simulink model "ARDroneTT"  (R2026a)
settings: Solver=ode1  StopTime=inf  FixedStep=sampleTime  EnableMultiTasking=on
values from neighbouring files (symbols this model uses):
  sampleTime = 0.03    [setupHover.m]    (also in setupTT.m; setupWPTracking.m = 0.065)
undefined symbols (not defined in the file or in its folder): DiscIntNeverNeededParam, Standard_Devices, UDP_Protocol
libraries: sldrtlib x3, dspnetwork x3, ARBlocks x2, simulink x1, aerolibanimutils x1
settings Model: ExtModeTrigDuration=100000  Creator=Paul  LastModifiedBy=dasos
settings DataIOCC: SignalLoggingSaveFormat=ModelDataLogs  TimeSaveName=time
settings OptimizationCC: InitFltsAndDblsToZero=on
settings DebuggingCC: UnderspecifiedInitializationDetection=Classic
settings HardwareCC: ProdBitPerLong=64.0  ProdHWDeviceType=Intel->x86-64 (Linux 64)
settings RTWCC: SystemTargetFile=sldrt.tlc  TemplateMakefile=sldrt.tmf  RTWCompilerOptimization=on  Description=Simulink Desktop Real-Time
settings CodeAppCC: MaxIdLength=95.0
settings SimulinkDesktopRealTimeCC: RealTimeExecution=kernel  ExtModeTransport=0.0  ExtModeStaticAllocSize=1000000.0  TargetLibSuffix=_sldrt.a  TargetPreCompLibLocation=C:\Program Files\MATLAB\R2026a\toolbox\sldrt\lib\win64  TargetLangStandard=C89/C90 (ANSI)  MultiwordLength=2048.0  ParMdlRefBuildCompliant=on

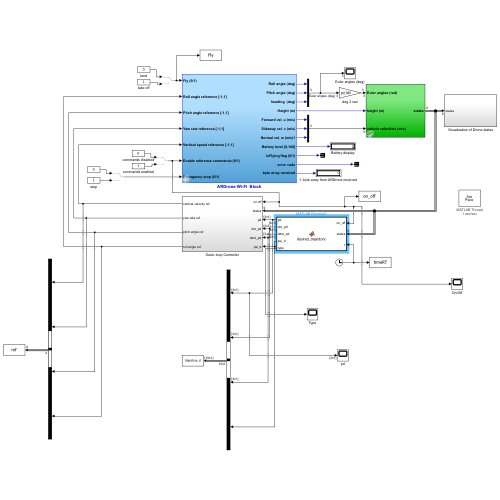
[thumbnail: Simulink's stored preview of the top-level diagram]
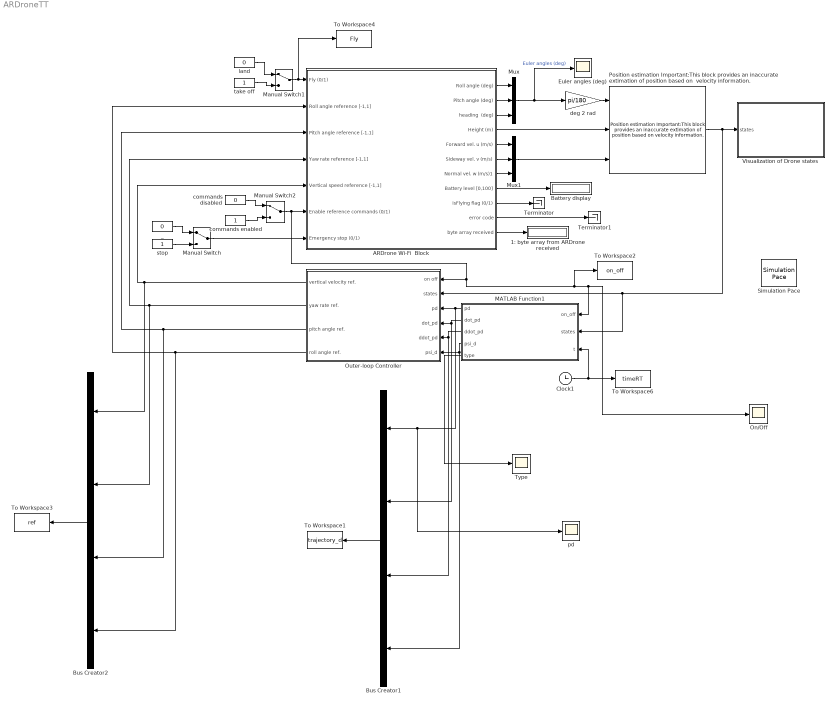
== system ARDroneTT ==
  "1: byte array from ARDrone received " : Display
  ARDrone Wi-Fi  Block : Subsystem  AncestorBlock="ARBlocks/ARDrone Wi-Fi  Block"
  Battery display : Display
  Bus Creator1 : BusCreator  Inputs=4
  Bus Creator2 : BusCreator  Inputs=4
  Clock1 : Clock
  Euler angles (deg) : Scope
      settings: ActiveDisplayYMinimum=-189.44824826717377  ActiveDisplayYMaximum=31.394250273704525  DataLoggingMaxPoints=500000
  MATLAB Function1 : MATLAB Function  TreatAsAtomicUnit=on  SystemSampleTime=sampleTime
  Manual Switch : ManualSwitch
  Manual Switch1 : ManualSwitch
  Manual Switch2 : ManualSwitch
  Mux : Mux  Inputs=3
  Mux1 : Mux  Inputs=3
  On/Off : Scope
      settings: ActiveDisplayYMinimum=-0.12499999999999997  ActiveDisplayYMaximum=1.125  DataLoggingMaxPoints=500000  DataLoggingVariableName=ScopeData13
  Outer-loop Controller : Subsystem
  "Position estimation Important:This block provides an inaccurate extimation of position based on  velocity information. " : ARBlocks/Position estimation Important:This block provides an  inaccurate extimation of position  based on  velocity information.   SystemSampleTime=-1  VariantActivationTime=update diagram  EmptyChoice=off  PassThrough=off  PassThroughVariantControl=(default)  EmptyChoiceVariantControl=(default)  AllowFlexibleInterface=on  Latency=0  AutoFrameSizeCalculation=off
  Simulation Pace : aerolibanimutils/Simulation Pace  SimulationPace=1  SleepMode=MATLAB Thread  OutputPaceError=off  SampleTime=sampleTime
  Terminator : Terminator
  Terminator1 : Terminator
  To Workspace1 : ToWorkspace  VariableName=trajectory_d  SampleTime=sampleTime
  To Workspace2 : ToWorkspace  VariableName=on_off  SampleTime=sampleTime
  To Workspace3 : ToWorkspace  VariableName=ref  SampleTime=sampleTime
  To Workspace4 : ToWorkspace  VariableName=Fly  SampleTime=sampleTime
  To Workspace6 : ToWorkspace  VariableName=timeRT  SampleTime=sampleTime
  Type : Scope
      settings: ActiveDisplayYMinimum=-1.25  ActiveDisplayYMaximum=1.25  DataLoggingMaxPoints=500000  DataLoggingVariableName=ScopeData12
  Visualization of Drone states : Subsystem
  _ : Constant  Value=0
  commands disabled : Constant  Value=0
  commands enabled : Constant
  deg 2 rad : Gain  Gain=pi/180
  land : Constant  Value=0
  pd : Scope
      settings: ActiveDisplayYMinimum=-1.25  ActiveDisplayYMaximum=1.25  DataLoggingMaxPoints=500000  DataLoggingVariableName=ScopeData11
  stop : Constant
  take off : Constant
  wires:
  _/1 -> Manual Switch/1
  stop/1 -> Manual Switch/2
  land/1 -> Manual Switch1/1
  take off/1 -> Manual Switch1/2
  commands disabled/1 -> Manual Switch2/1
  commands enabled/1 -> Manual Switch2/2
  Manual Switch1/1 -> To Workspace4/1, ARDrone Wi-Fi  Block/1(Fly (0/1))
  Manual Switch2/1 -> ARDrone Wi-Fi  Block/6(Enable reference commands (0/1)), To Workspace2/1, On/Off/1, MATLAB Function1/1(on_off), Outer-loop Controller/1(on off)
  Manual Switch/1 -> ARDrone Wi-Fi  Block/7(Emergency stop (0/1))
  ARDrone Wi-Fi  Block/1(Roll angle (deg)) -> Mux/1
  ARDrone Wi-Fi  Block/2(Pitch angle (deg)) -> Mux/2
  ARDrone Wi-Fi  Block/5(Forward vel. u (m/s)) -> Mux1/1
  ARDrone Wi-Fi  Block/6(Sideway vel. v (m/s)) -> Mux1/2
  ARDrone Wi-Fi  Block/7(Normal vel. w (m/s)1) -> Mux1/3
  Mux/1 -> Euler angles (deg)/1, deg 2 rad/1  "Euler angles (deg)"
  ARDrone Wi-Fi  Block/8(Battery level [0,100]) -> Battery display/1
  "Position estimation Important:This block provides an inaccurate extimation of position based on  velocity information. "/1 -> MATLAB Function1/2(states), Outer-loop Controller/2(states), Visualization of Drone states/1(states)
  deg 2 rad/1 -> "Position estimation Important:This block provides an inaccurate extimation of position based on  velocity information. "/1
  ARDrone Wi-Fi  Block/4(Height (m)) -> "Position estimation Important:This block provides an inaccurate extimation of position based on  velocity information. "/2
  Mux1/1 -> "Position estimation Important:This block provides an inaccurate extimation of position based on  velocity information. "/3
  ARDrone Wi-Fi  Block/3(heading  (deg)) -> Mux/3
  ARDrone Wi-Fi  Block/9(isFlying flag (0/1)) -> Terminator/1
  ARDrone Wi-Fi  Block/10(error code) -> Terminator1/1
  ARDrone Wi-Fi  Block/11(byte array received) -> "1: byte array from ARDrone received "/1
  Clock1/1 -> MATLAB Function1/3(t), To Workspace6/1
  MATLAB Function1/1(pd) -> pd/1, Bus Creator1/1, Outer-loop Controller/3(pd)
  MATLAB Function1/2(dot_pd) -> Bus Creator1/2, Outer-loop Controller/4(dot_pd)
  MATLAB Function1/3(ddot_pd) -> Bus Creator1/3, Outer-loop Controller/5(ddot_pd)
  MATLAB Function1/4(psi_d) -> Bus Creator1/4, Outer-loop Controller/6(psi_d)
  Bus Creator1/1 -> To Workspace1/1
  Outer-loop Controller/3(pitch angle ref.) -> Bus Creator2/3, ARDrone Wi-Fi  Block/3(Pitch angle reference [-1,1])
  Outer-loop Controller/2(yaw rate ref.) -> Bus Creator2/2, ARDrone Wi-Fi  Block/4(Yaw rate reference [-1,1])
  Outer-loop Controller/4(roll angle ref.) -> Bus Creator2/4, ARDrone Wi-Fi  Block/2(Roll angle reference [-1,1])
  Outer-loop Controller/1(vertical velocity ref.) -> Bus Creator2/1, ARDrone Wi-Fi  Block/5(Vertical speed reference [-1,1])
  Bus Creator2/1 -> To Workspace3/1
  MATLAB Function1/5(type) -> Type/1

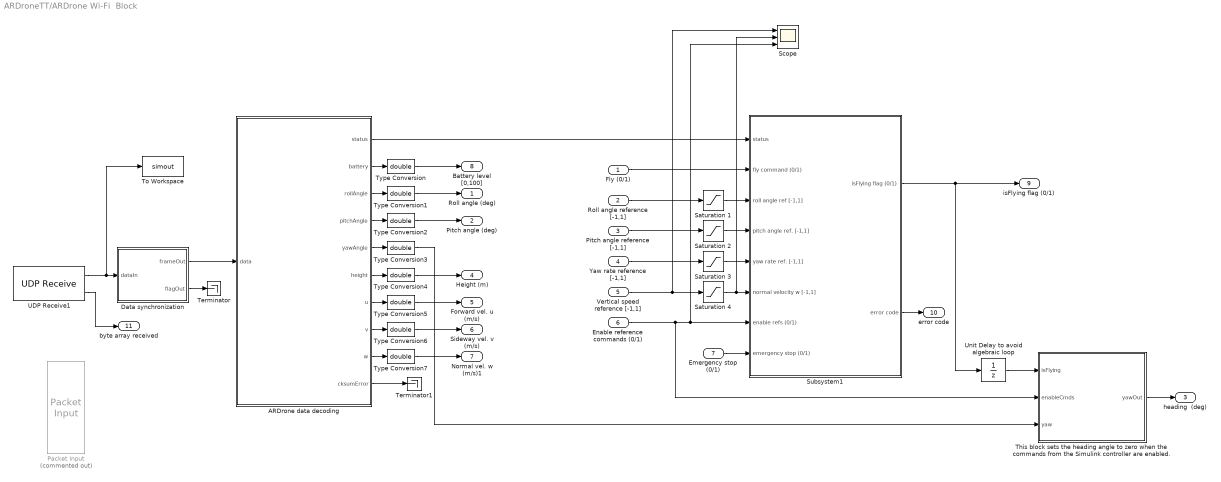
== system ARDroneTT/ARDrone Wi-Fi  Block ==
  Fly (0/1) : Inport
  Roll angle reference [-1,1] : Inport  Port=2
  Pitch angle reference [-1,1] : Inport  Port=3
  Yaw rate reference [-1,1] : Inport  Port=4
  Vertical speed reference [-1,1] : Inport  Port=5
  Enable reference commands (0/1) : Inport  Port=6
  Emergency stop (0/1) : Inport  Port=7
  ARDrone data decoding : MATLAB Function  TreatAsAtomicUnit=on
  "Data synchronization " : MATLAB Function  TreatAsAtomicUnit=on
  Packet Input : sldrtlib/Packet Input  Commented=on  SampleTime=sampleTime  MaxMissedTicks=100  ShowMissedTicks=off  YieldWhenWaiting=off  DrvName=Standard_Devices/UDP_Protocol  DrvAddress=5554  DrvOptions=[3232235777 5554]  PacketSize=500  DataTypes='500*uint8'  ShowReady=on  ShowError=off  PacketID=1  ByteOrder=1  ShowTimestamp=off
      settings: AttributesFormatString=UDP Protocol [5554]
  Saturation 1 : Saturate  UpperLimit=1  LowerLimit=-1
  Saturation 2 : Saturate  UpperLimit=1  LowerLimit=-1
  Saturation 3 : Saturate  UpperLimit=1  LowerLimit=-1
  Saturation 4 : Saturate  UpperLimit=1.5  LowerLimit=-1.5
  Scope : Scope  NumInputPorts=3
      settings: ActiveDisplayYMinimum=-0.2465  ActiveDisplayYMaximum=1.1385  DataLoggingVariableName=ScopeData2
  Subsystem1 : Subsystem
  Terminator : Terminator
  Terminator1 : Terminator
  "This block sets the heading angle to zero when the commands from the Simulink controller are enabled. " : MATLAB Function  TreatAsAtomicUnit=on
  To Workspace : ToWorkspace  VariableName=simout  SampleTime=-1
  Type Conversion{,1..7} (8 alike) : DataTypeConversion  OutDataTypeStr=double  SaturateOnIntegerOverflow=off  RndMeth=Floor
  UDP Receive1 : dspnetwork/UDP Receive  localURL='0.0.0.0'  localPort=5554  remoteURL='192.168.1.1'  remotePort=-1  recvBufferSize=8192  dims=500  signalDatatype=uint8  isComplex=off  isVarSize=off  showBlockingTime=off  blockingTime=0  sampletime=sampleTime  blockPlatform=[]
  Unit Delay to avoid algebraic loop : UnitDelay  SampleTime=-1
  Roll angle (deg) : Outport  VectorParamsAs1DForOutWhenUnconnected=off
  Pitch angle (deg) : Outport  Port=2  VectorParamsAs1DForOutWhenUnconnected=off
  heading  (deg) : Outport  Port=3  VectorParamsAs1DForOutWhenUnconnected=off
  Height (m) : Outport  Port=4  VectorParamsAs1DForOutWhenUnconnected=off
  Forward vel. u (m/s) : Outport  Port=5  VectorParamsAs1DForOutWhenUnconnected=off
  Sideway vel. v (m/s) : Outport  Port=6  VectorParamsAs1DForOutWhenUnconnected=off
  Normal vel. w (m/s)1 : Outport  Port=7  VectorParamsAs1DForOutWhenUnconnected=off
  Battery level [0,100] : Outport  Port=8  VectorParamsAs1DForOutWhenUnconnected=off
  isFlying flag (0/1) : Outport  Port=9  VectorParamsAs1DForOutWhenUnconnected=off
  error code : Outport  Port=10  VectorParamsAs1DForOutWhenUnconnected=off
  byte array received : Outport  Port=11  VectorParamsAs1DForOutWhenUnconnected=off
  wires:
  Unit Delay to avoid algebraic loop/1 -> "This block sets the heading angle to zero when the commands from the Simulink controller are enabled. "/1(isFlying)
  "Data synchronization "/2(flagOut) -> Terminator/1
  Saturation 4/1 -> Scope/2, Subsystem1/6(normal velocity w [-1,1])
  Saturation 3/1 -> Subsystem1/5(yaw rate ref. [-1,1])
  Saturation 2/1 -> Subsystem1/4(pitch angle ref. [-1,1])
  Saturation 1/1 -> Subsystem1/3(roll angle ref [-1,1])
  Fly (0/1)/1 -> Subsystem1/2(fly command (0/1))
  "This block sets the heading angle to zero when the commands from the Simulink controller are enabled. "/1(yawOut) -> heading  (deg)/1
  Type Conversion3/1 -> "This block sets the heading angle to zero when the commands from the Simulink controller are enabled. "/3(yaw)
  Type Conversion7/1 -> Normal vel. w (m/s)1/1
  Type Conversion6/1 -> Sideway vel. v (m/s)/1
  Type Conversion5/1 -> Forward vel. u (m/s)/1
  Type Conversion4/1 -> Height (m)/1
  Type Conversion2/1 -> Pitch angle (deg)/1
  Type Conversion1/1 -> Roll angle (deg)/1
  Type Conversion/1 -> Battery level [0,100]/1
  ARDrone data decoding/10(cksumError) -> Terminator1/1
  Subsystem1/2(error code) -> error code/1
  Subsystem1/1(isFlying flag (0/1)) -> isFlying flag (0/1)/1, Unit Delay to avoid algebraic loop/1
  Emergency stop (0/1)/1 -> Subsystem1/8(emergency stop (0/1))
  Enable reference commands (0/1)/1 -> Scope/3, Subsystem1/7(enable refs (0/1)), "This block sets the heading angle to zero when the commands from the Simulink controller are enabled. "/2(enableCmds)
  Vertical speed reference [-1,1]/1 -> Scope/1, Saturation 4/1
  Yaw rate reference [-1,1]/1 -> Saturation 3/1
  Pitch angle reference [-1,1]/1 -> Saturation 2/1
  Roll angle reference [-1,1]/1 -> Saturation 1/1
  ARDrone data decoding/1(status) -> Subsystem1/1(status)
  UDP Receive1/2 -> byte array received/1
  ARDrone data decoding/9(w) -> Type Conversion7/1
  ARDrone data decoding/8(v) -> Type Conversion6/1
  ARDrone data decoding/7(u) -> Type Conversion5/1
  ARDrone data decoding/4(pitchAngle) -> Type Conversion2/1
  ARDrone data decoding/3(rollAngle) -> Type Conversion1/1
  ARDrone data decoding/6(height) -> Type Conversion4/1
  ARDrone data decoding/2(battery) -> Type Conversion/1
  ARDrone data decoding/5(yawAngle) -> Type Conversion3/1
  "Data synchronization "/1(frameOut) -> ARDrone data decoding/1(data)
  UDP Receive1/1 -> To Workspace/1, "Data synchronization "/1(dataIn)

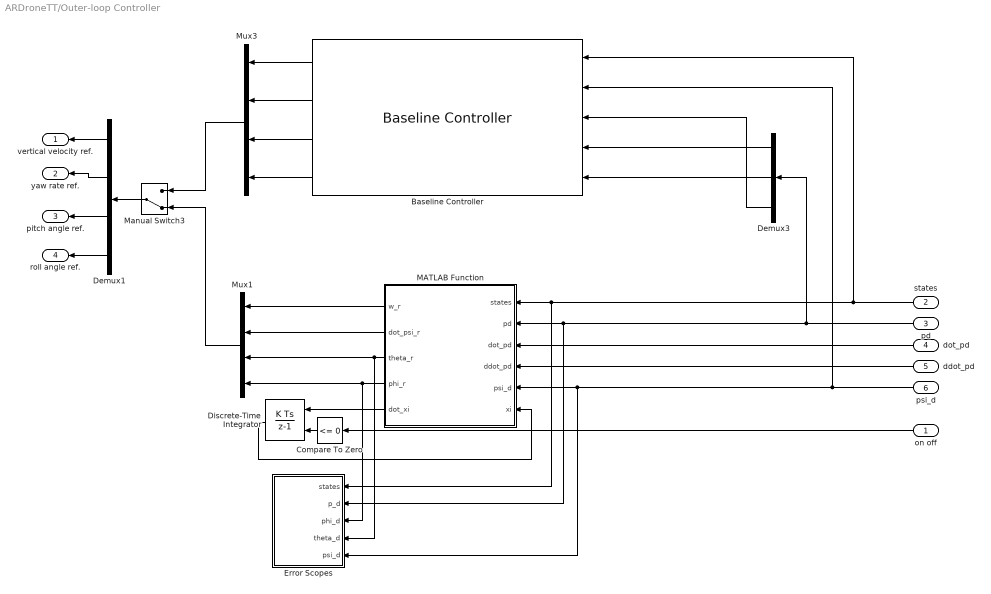
== system ARDroneTT/Outer-loop Controller ==
  on off : Inport  PortDimensions=1
  states : Inport  Port=2
  pd : Inport  Port=3  PortDimensions=[3 1]
  dot_pd : Inport  Port=4  PortDimensions=[3 1]
  ddot_pd : Inport  Port=5  PortDimensions=[3 1]
  psi_d : Inport  Port=6  PortDimensions=1
  Baseline Controller : ARBlocks/Baseline Controller  SystemSampleTime=-1  VariantActivationTime=update diagram  EmptyChoice=off  PassThrough=off  PassThroughVariantControl=(default)  EmptyChoiceVariantControl=(default)  AllowFlexibleInterface=on  Latency=0  AutoFrameSizeCalculation=off
  Compare To Zero : simulink/Logic and Bit Operations/Compare To Zero  relop=<=  OutDataTypeStr=boolean
  Demux1 : Demux  Outputs=[1,1,1,1]
  Demux3 : Demux  Outputs=[1,1,1]
  Discrete-Time Integrator : DiscreteIntegrator  ExternalReset=level  InitialCondition=[0;0;0;0]  SampleTime=sampleTime  UpperSaturationLimit=10  LowerSaturationLimit=-10  ICPrevOutput=DiscIntNeverNeededParam  ICPrevScaledInput=DiscIntNeverNeededParam
  Error Scopes : Subsystem
  MATLAB Function : MATLAB Function  TreatAsAtomicUnit=on  SystemSampleTime=sampleTime
  Manual Switch3 : ManualSwitch  CurrentSetting=0
  Mux1 : Mux  Inputs=[1,1,1,1]
  Mux3 : Mux  Inputs=[1,1,1,1]
  vertical velocity ref. : Outport  VectorParamsAs1DForOutWhenUnconnected=off
  yaw rate ref. : Outport  Port=2  VectorParamsAs1DForOutWhenUnconnected=off
  pitch angle ref. : Outport  Port=3  VectorParamsAs1DForOutWhenUnconnected=off
  roll angle ref. : Outport  Port=4  VectorParamsAs1DForOutWhenUnconnected=off
  wires:
  states/1 -> Baseline Controller/1, Error Scopes/1(states), MATLAB Function/1(states)
  MATLAB Function/1(w_r) -> Mux1/1
  MATLAB Function/3(theta_r) -> Mux1/3, Error Scopes/4(theta_d)
  MATLAB Function/4(phi_r) -> Mux1/4, Error Scopes/3(phi_d)
  MATLAB Function/2(dot_psi_r) -> Mux1/2
  MATLAB Function/5(dot_xi) -> Discrete-Time Integrator/1
  Discrete-Time Integrator/1 -> MATLAB Function/6(xi)
  pd/1 -> Demux3/1, Error Scopes/2(p_d), MATLAB Function/2(pd)
  dot_pd/1 -> MATLAB Function/3(dot_pd)
  ddot_pd/1 -> MATLAB Function/4(ddot_pd)
  psi_d/1 -> Error Scopes/5(psi_d), MATLAB Function/5(psi_d), Baseline Controller/2
  Demux3/1 -> Baseline Controller/4
  Demux3/2 -> Baseline Controller/5
  Demux3/3 -> Baseline Controller/3
  Baseline Controller/4 -> Mux3/4
  Baseline Controller/3 -> Mux3/3
  Baseline Controller/2 -> Mux3/2
  Baseline Controller/1 -> Mux3/1
  Mux3/1 -> Manual Switch3/1
  Demux1/1 -> vertical velocity ref./1
  Demux1/2 -> yaw rate ref./1
  Demux1/3 -> pitch angle ref./1
  Demux1/4 -> roll angle ref./1
  Manual Switch3/1 -> Demux1/1
  Mux1/1 -> Manual Switch3/2
  on off/1 -> Compare To Zero/1
  Compare To Zero/1 -> Discrete-Time Integrator/2

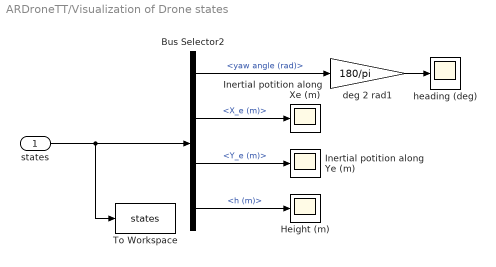
== system ARDroneTT/Visualization of Drone states ==
  states : Inport
  Bus Selector2 : BusSelector  OutputSignals=yaw angle (rad),X_e (m),Y_e (m),h (m)
  Height (m) : Scope
      settings: ActiveDisplayYMinimum=-0.13049999999999998  ActiveDisplayYMaximum=1.1745  DataLoggingMaxPoints=500000  DataLoggingVariableName=ScopeData5
  Inertial potition along Xe (m) : Scope
      settings: ActiveDisplayYMinimum=-1.1928531151622555  ActiveDisplayYMaximum=0.13253923501802836  DataLoggingMaxPoints=500000  DataLoggingVariableName=ScopeData3
  Inertial potition along Ye (m) : Scope
      settings: ActiveDisplayYMinimum=-0.61688622691602624  ActiveDisplayYMaximum=0.0717087724162803  DataLoggingMaxPoints=500000  DataLoggingVariableName=ScopeData4
  To Workspace : ToWorkspace  VariableName=states  SaveFormat=Structure With Time  SampleTime=-1
  deg 2 rad1 : Gain  Gain=180/pi
  heading (deg) : Scope
      settings: ActiveDisplayYMinimum=-22.5  ActiveDisplayYMaximum=22.5  DataLoggingMaxPoints=500000  DataLoggingVariableName=ScopeData2
  wires:
  states/1 -> To Workspace/1, Bus Selector2/1
  Bus Selector2/1 -> deg 2 rad1/1  "<yaw angle (rad)>"
  Bus Selector2/2 -> Inertial potition along Xe (m)/1  "<X_e (m)>"
  Bus Selector2/3 -> Inertial potition along Ye (m)/1  "<Y_e (m)>"
  Bus Selector2/4 -> Height (m)/1  "<h (m)>"
  deg 2 rad1/1 -> heading (deg)/1

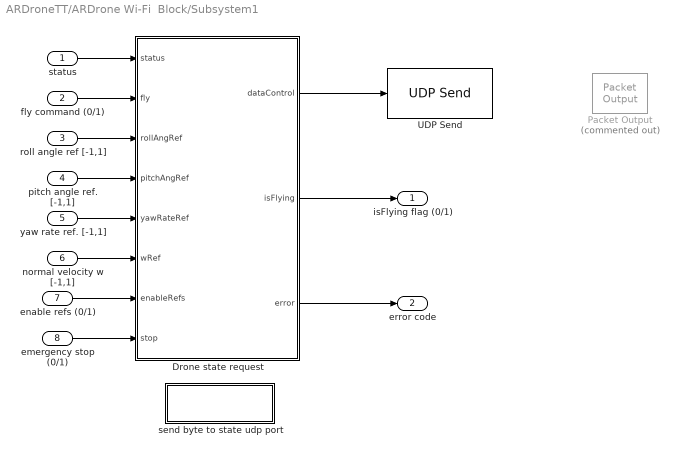
== system ARDroneTT/ARDrone Wi-Fi  Block/Subsystem1 ==
  status : Inport
  fly command (0/1) : Inport  Port=2
  roll angle ref [-1,1] : Inport  Port=3
  pitch angle ref. [-1,1] : Inport  Port=4
  yaw rate ref. [-1,1] : Inport  Port=5
  normal velocity w [-1,1] : Inport  Port=6
  enable refs (0/1) : Inport  Port=7
  emergency stop (0/1) : Inport  Port=8
  Drone state request : MATLAB Function  TreatAsAtomicUnit=on  SystemSampleTime=sampleTime
  Packet Output : sldrtlib/Packet Output  Commented=on  SampleTime=sampleTime*7  MaxMissedTicks=100  ShowMissedTicks=off  YieldWhenWaiting=off  DrvName=Standard_Devices/UDP_Protocol  DrvAddress=5556  DrvOptions=[3232235777 5556]  PacketSize=150  DataTypes='150*uint8'  ShowReady=off  ShowError=off  PacketID=1  ByteOrder=1  InitialValue=[]  FinalValue=[]
      settings: AttributesFormatString=UDP Protocol [5556]
  UDP Send : dspnetwork/UDP Send  remoteURL='192.168.1.1'  remotePort=5556  localURL='0.0.0.0'  localPortSource=Specify via dialog  localPort=5556  sendBufferSize=8192  sampletime=-1  blockPlatform=[]  separateLengthPort=0
  "send byte to state udp port " : Subsystem
  isFlying flag (0/1) : Outport  VectorParamsAs1DForOutWhenUnconnected=off
  error code : Outport  Port=2  VectorParamsAs1DForOutWhenUnconnected=off
  wires:
  Drone state request/3(error) -> error code/1
  emergency stop (0/1)/1 -> Drone state request/8(stop)
  enable refs (0/1)/1 -> Drone state request/7(enableRefs)
  normal velocity w [-1,1]/1 -> Drone state request/6(wRef)
  yaw rate ref. [-1,1]/1 -> Drone state request/5(yawRateRef)
  roll angle ref [-1,1]/1 -> Drone state request/3(rollAngRef)
  Drone state request/2(isFlying) -> isFlying flag (0/1)/1
  status/1 -> Drone state request/1(status)
  pitch angle ref. [-1,1]/1 -> Drone state request/4(pitchAngRef)
  fly command (0/1)/1 -> Drone state request/2(fly)
  Drone state request/1(dataControl) -> UDP Send/1

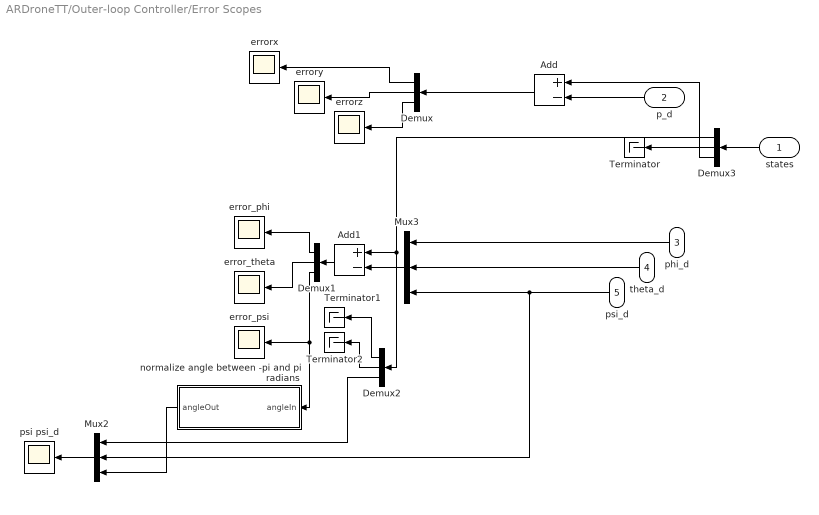
== system ARDroneTT/Outer-loop Controller/Error Scopes ==
  states : Inport
  p_d : Inport  Port=2
  phi_d : Inport  Port=3
  theta_d : Inport  Port=4
  psi_d : Inport  Port=5
  Add : Sum  Inputs=+-
  Add1 : Sum  Inputs=+-
  Demux : Demux  Outputs=3
  Demux1 : Demux  Outputs=[1,1,1]
  Demux2 : Demux  Outputs=[1,1,1]
  Demux3 : Demux  Outputs=[3,3,3]
  Mux2 : Mux  Inputs=[1,1,1]
  Mux3 : Mux  Inputs=[1,1,1]
  Terminator : Terminator
  Terminator1 : Terminator
  Terminator2 : Terminator
  error_phi : Scope
      settings: ActiveDisplayYMinimum=-0.10055  ActiveDisplayYMaximum=0.0129  DataLoggingMaxPoints=500000  DataLoggingVariableName=ScopeData8
  error_psi : Scope
      settings: ActiveDisplayYMinimum=-0.01923  ActiveDisplayYMaximum=0.00214  DataLoggingMaxPoints=500000  DataLoggingVariableName=ScopeData10
  error_theta : Scope
      settings: ActiveDisplayYMinimum=-0.0733  ActiveDisplayYMaximum=0.55697  DataLoggingMaxPoints=500000  DataLoggingVariableName=ScopeData9
  errorx : Scope
      settings: ActiveDisplayYMinimum=-0.75254  ActiveDisplayYMaximum=0.08362  DataLoggingMaxPoints=500000  DataLoggingVariableName=ScopeData6
  errory : Scope
      settings: ActiveDisplayYMinimum=-101.73315  ActiveDisplayYMaximum=11.30368  DataLoggingMaxPoints=500000
  errorz : Scope
      settings: ActiveDisplayYMinimum=-1.12689  ActiveDisplayYMaximum=0.14199  DataLoggingMaxPoints=500000  DataLoggingVariableName=ScopeData7
  normalize angle between -pi and pi radians : MATLAB Function  TreatAsAtomicUnit=on
  psi psi_d : Scope
      settings: ActiveDisplayYMinimum=-0.25025  ActiveDisplayYMaximum=0.25226  DataLoggingMaxPoints=500000  DataLoggingVariableName=psi
  wires:
  Add/1 -> Demux/1
  Demux/1 -> errorx/1
  Demux/3 -> errorz/1
  Demux/2 -> errory/1
  Demux1/1 -> error_phi/1
  Demux1/2 -> error_theta/1
  p_d/1 -> Add/2
  phi_d/1 -> Mux3/1
  theta_d/1 -> Mux3/2
  psi_d/1 -> Mux2/2, Mux3/3
  Mux2/1 -> psi psi_d/1
  Demux1/3 -> normalize angle between -pi and pi radians/1(angleIn), error_psi/1
  Demux2/3 -> Mux2/1
  normalize angle between -pi and pi radians/1(angleOut) -> Mux2/3
  states/1 -> Demux3/1
  Demux3/3 -> Add/1
  Demux3/1 -> Add1/1, Demux2/1
  Add1/1 -> Demux1/1
  Mux3/1 -> Add1/2
  Demux3/2 -> Terminator/1
  Demux2/1 -> Terminator1/1
  Demux2/2 -> Terminator2/1

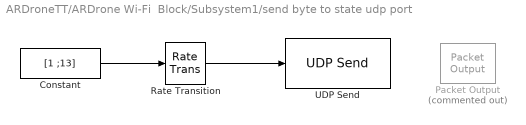
== system ARDroneTT/ARDrone Wi-Fi  Block/Subsystem1/send byte to state udp port  ==
  Constant : Constant  Value=[1 ;13]  OutDataTypeStr=uint8
  Packet Output : sldrtlib/Packet Output  Commented=on  SampleTime=sampleTime*10  MaxMissedTicks=100  ShowMissedTicks=off  YieldWhenWaiting=off  DrvName=Standard_Devices/UDP_Protocol  DrvAddress=5554  DrvOptions=[3232235777 5554]  PacketSize=2  DataTypes='2*uint8'  ShowReady=off  ShowError=off  PacketID=1  ByteOrder=1  InitialValue=[]  FinalValue=[]
      settings: AttributesFormatString=UDP Protocol [5554]
  Rate Transition : RateTransition
  UDP Send : dspnetwork/UDP Send  remoteURL='192.168.1.1'  remotePort=5554  localURL='0.0.0.0'  localPortSource=Specify via dialog  localPort=5554  sendBufferSize=8192  sampletime=-1  blockPlatform=[]  separateLengthPort=0
  wires:
  Constant/1 -> Rate Transition/1
  Rate Transition/1 -> UDP Send/1

== matlab function ARDroneTT/ARDrone Wi-Fi  Block/Subsystem1/Drone state request ==
  data: status input; fly input; rollAngRef input; pitchAngRef input; yawRateRef input; wRef input; enableRefs input; dataControl output; isFlying output; stop input; error output
function [dataControl, isFlying, error] = fcn( status, fly, rollAngRef, pitchAngRef, yawRateRef, wRef, enableRefs, stop)
%#codegen

% Persistent variables.
persistent SequenceNumber ;

% Initialization of persistent variables at first time step. 

if isempty(SequenceNumber)
    SequenceNumber = 1 ;
end



% Error code / No error: 0
error=0;

% Boolean of flying status / Flying: 1
isFlying = status(32) ;

% Byte array of size 150 to be sent to the drone.
strOut = uint8(zeros(150,1)) ;

% String that coontains a variable size command. 
% cmd is concatenated with previous commands at each sample
cmd = '';

% At first time step and every 100 time steps, data is requested.
if (SequenceNumber <=1 || mod(SequenceNumber, 100) ==0 )
    SequenceNumber = SequenceNumber+1; 
    strCmd = getString(SequenceNumber) ;
    cmd = ['AT*CONFIG=' strCmd ',"general:navdata_demo","TRUE"' char(13)];
    
end

SequenceNumber = SequenceNumber+1;
strCmd = getString(SequenceNumber) ;
cmd = [cmd 'AT*COMWDG=' strCmd char(13)];


if stop ==1 % Emergency stop
   cmd = ['AT*REF=' strCmd ',290717952' char(13)] ; 
    
else % Not emergency stop
    
    if SequenceNumber >20 && SequenceNumber <22
        
        % Trim vehicle state estimation / angles set to zero
        SequenceNumber =SequenceNumber+1;
        strCmd = getString(SequenceNumber) ;
        cmd = [cmd 'AT*FTRIM=' strCmd char(13)] ;
        
    elseif SequenceNumber >=22 && SequenceNumber <25
        cmd = [cmd 'AT*CONFIG=' strCmd '"conrol:altitude_max","100000"' char(13)] ;
        
        
    elseif SequenceNumber >=25
        
        if ( fly == 1  )
            
            if (isFlying ==0)
                
                SequenceNumber =SequenceNumber+1;
                strCmd = getString(SequenceNumber) ;
                cmd = [cmd 'AT*REF=' strCmd ',290718208' char(13)] ;
            
            elseif isFlying==1 && enableRefs==1
                
                SequenceNumber =SequenceNumber+1;
                strCmd = getString(SequenceNumber) ;
                      
                cmd = [cmd 'AT*PCMD=' strCmd ',1,'] ;
                 
                aux = double (float2IEEE754 (rollAngRef) )  ;
                strAux = getString(abs(aux)) ; 
                if rollAngRef<0
                   strAux = [char(45) strAux] ; 
                end
                cmd = [cmd strAux ','];
                      
               aux = double (float2IEEE754 (pitchAngRef) ) ;
               strAux = getString(abs(aux)) ; 
               if pitchAngRef<0
                    strAux = [char(45) strAux] ; 
               end
               cmd = [cmd strAux ','];
                      
               aux =  double(float2IEEE754 (wRef)) ;
               strAux = getString(abs(aux)) ; 
               if wRef<0
                    strAux = [char(45) strAux] ; 
               end
               cmd = [cmd strAux ','];
                      
                      
               aux =  double (float2IEEE754 (yawRateRef) ) ;
               strAux = getString(abs(aux)) ; 
               if yawRateRef <0
                     error=2; 
                     strAux = [char(45) strAux] ; 
               end
               cmd = [cmd strAux char(13)];
               
                
            end
            
            
        elseif ( fly==0 )
                
               if isFlying ==1
                    SequenceNumber =SequenceNumber+1;
                    strCmd = getString(SequenceNumber) ;
                    cmd = [cmd 'AT*REF=' strCmd ',290717696' char(13)] ;
                    
              end
        end
        
    end
    
    
    
end

% cmd must contain less than 150 bytes. 
if (length(cmd)<150)
    strOut(1:length(cmd)) = cmd ;
else
    error =1; 
end

dataControl = strOut;

end


%% My str2num function that allows for code generation
function [ strOut] = getString( a )
d=1;

if (a<10)
    d=1;
end

if (a >=10 && a <100)
    d=2;
end

if (a >=100 && a <1000)
    d=3;
end

if (a >=1000 && a <10000)
    d=4;
end

if (a >=10000 && a <100000)
    d=5;
end

if (a >=100000 && a <1000000)
    d=6;
end

if (a >=1000000 && a <10000000)
    d=7;
end

if (a >=10000000 && a <100000000)
    d=8;
end

if (a >=100000000 && a <1000000000)
    d=9;
end

if (a >=1000000000 && a <10000000000)
    d=10;
end

if (a >=10000000000 )
    d=11;
end



digit = uint8(zeros(1,d)) ;
resTotal = 0;
%d = length(a) ;
for k=1:d
    
    res1 = mod(a,10^k)/(10^(k-1)) ;
    %( mod(a,10*k) - resTotal)/(10*k) ;
    
    digit(d-k+1) = char(48 + res1);
    resTotal = (10^(k-1))*res1 +resTotal;
    
end

strOut = char(digit) ;


end

%% Function to obtain a IEEE754 representation of a float number
function [ iVal ] = float2IEEE754( fVal )

binData = dec2bin(typecast (single(fVal), 'uint8'),8);

binData2 =[ binData(4,:) binData(3,:) binData(2,:) binData(1,:)];
iVal =0; 
for k=32:-1:1
    
    if (binData2(k) =='1')
        bit = 1;
    else
        bit =0;
    end
    
    if k == 1
        iVal = iVal - bit*2^(31);
    else
        iVal = iVal + bit*2^(32-k) ; 
    end
    
end

iVal = int32(iVal);

end

== matlab function ARDroneTT/ARDrone Wi-Fi  Block/ARDrone data decoding ==
  data: status output; battery output; rollAngle output; pitchAngle output; data input; yawAngle output; height output; u output; v output; w output; cksumError output
function [ status, battery,  rollAngle, pitchAngle, yawAngle, height, u,v,w , cksumError ]= fcn(data)
%#codegen

% Checksum array. cksum(1) contains the computed checksum, cksum(2)
% contains the checksum sent by the ARDrone. 
cksum = [0 0 ]; 

% Previous value of height 
persistent hPrev ; 
% Previous data packet
persistent dataPrev ; 

% Initialization of persistent variables
if isempty(hPrev)
    hPrev=0 ; 
end

if isempty(dataPrev)
    dataPrev = uint8(zeros(496,1)) ;
end

% Computing checksum
cksum(1) =  sum(double(data(1:end-8))) +442; 
% Checksum given by the drone
cksum(2) = double(data(end-3)) + double(data(end-2))*256 +  double(data(end-1))*256^2 + double(data(end))*256^3 ; 
% Checksum error
cksumError = abs(cksum(1)-cksum(2));
%% Change the following if statement to ensure that the data checksum is valid 
%if (data(15) == 148 && cksumError==0 )
if (data(15) == 148  )
    dataPrev = data; 
else
    data = dataPrev; 
end

% Converting bytes to drone information
status = getDroneState(data(1:4));
battery = decode(data(21:24),1); % unit: deg
pitchAngle = decode(data(25:28),0)/1000; % unit: deg
rollAngle = decode(data(29:32),0)/1000; % unit: deg
yawAngle = decode(data(33:36),0)/1000; % unit: deg
height = double(decode(data(37:40),1))/1000; % unit: deg
u = decode(data(41:44),0)/1000; % unit: m/s
v = decode(data(45:48),0)/1000; % unit: m/s
w = decode(data(49:52),0)/1000; % unit: m/s



if (status(32) ==1 && height< 0.2   )
    height = hPrev;
elseif status(32)==1 
    hPrev= height; 
end
  
    
end


function res = decode(input, mark)
% if mark = 1; then output a int
% else output the float value which is defined by SDK description.
% the input is an array (1*4) 
% e.g. : NDS(Battery_OS:Battery_OS+data_length-1)
%    hex_value = dec2hex(input);
%    hex_value = [hex_value(4,:),hex_value(3,:),hex_value(2,:),hex_value(1,:)];
    if mark ==1
        res = typecast(input,'uint32')%hex2num(hex_value);
    else
        res = typecast(input,'single'); %res = typecast(uint32(hex2dec(hex_value)),'single');
    end
    res = res(1);
end

function bin = getDroneState(input)
    bin = zeros(32,1); 
    hex = dec2hex(input);
    % put the hex_value in the order [31, 30......0]
    hex = [hex(4,:),hex(3,:),hex(2,:),hex(1,:)];
for i=1:length(hex)
    if hex(i)=='F'
        bin((i*4)-3:i*4)=[1 1 1 1];
    elseif hex(i)=='E'
        bin((i*4)-3:i*4)=[1 1 1 0];
    elseif hex(i)=='D'
        bin((i*4)-3:i*4)=[1 1 0 1];
    elseif hex(i)=='C'
        bin((i*4)-3:i*4)=[1 1 0 0];
    elseif hex(i)=='B'
        bin((i*4)-3:i*4)=[1 0 1 1];
    elseif hex(i)=='A'
        bin((i*4)-3:i*4)=[1 0 1 0];
    elseif hex(i)=='9'
        bin((i*4)-3:i*4)=[1 0 0 1];
    elseif hex(i)=='8'
        bin((i*4)-3:i*4)=[1 0 0 0];
    elseif hex(i)=='7'
        bin((i*4)-3:i*4)=[0 1 1 1];
    elseif hex(i)=='6'
        bin((i*4)-3:i*4)=[0 1 1 0];
    elseif hex(i)=='5'
        bin((i*4)-3:i*4)=[0 1 0 1];
    elseif hex(i)=='4'
        bin((i*4)-3:i*4)=[0 1 0 0];
    elseif hex(i)=='3'
        bin((i*4)-3:i*4)=[0 0 1 1];
    elseif hex(i)=='2'
        bin((i*4)-3:i*4)=[0 0 1 0];
    elseif hex(i)=='1'
        bin((i*4)-3:i*4)=[0 0 0 1];
    elseif hex(i)=='0'
        bin((i*4)-3:i*4)=[0 0 0 0];
    end
end

end

== matlab function ARDroneTT/ARDrone Wi-Fi  Block/Data synchronization  ==
  data: dataIn input; frameOut output; flagOut output
function [frameOut,flagOut]  = fcn(dataIn)
%#eml
%% Author: David Escobar Sanabria
%  Description: This function synchronizes data coming from the flight computer
%  computer. 
%  frameOut: Organized frame
%  frameIn: sequence of bytes not sync.
persistent frame; 
persistent lastFrame; 
persistent count; 
persistent countHeader; 
persistent countBuffer; 
persistent buffer; 

%% Size of byte array containing the data
sizePayload= 496;

%% Size of the array read each time step
nBytes = 500 ;%size(dataIn,1); 


%%%%%%%%%%%%%%%%%%%%%%%%%%%%%%%%%%%%%%%%%%%%%%%%%%%%%%%
%% Initialization of presistent variables
if isempty(buffer)
    buffer=uint8(zeros(1024,1));
end

if isempty(countBuffer)
    countBuffer=0;
end


if isempty(frame)
    frame=uint8(zeros(sizePayload,1));
end

if isempty(lastFrame)
    lastFrame=uint8(zeros(sizePayload,1));
end


if isempty(count)
    count=0;
end

if isempty(countHeader)
    countHeader=0;
end
%%%%%%%%%%%%%%%%%%%%%%%%%%%%%%%%%%%%%%%%%%%%%%%%%%%%%%%

%% Filling the buffer
buffer(countBuffer+1:countBuffer+nBytes) = dataIn;

bytesToRead = countBuffer+nBytes; 

%%%%%%%%%%%%%%%%%%%%%%%%%%%%%%%%%%%%%%%%%%%%%%%%%%%%%%%
%% Reading buffer

for k=1:bytesToRead    
    if(countHeader==4 && count<sizePayload)
        bytesLeft = sizePayload-count;
        frame(count+1:sizePayload) = buffer(k:k+bytesLeft-1);
        count = sizePayload;
        countBuffer = bytesToRead-bytesLeft ;
        buffer(1:countBuffer) = buffer(k+bytesLeft:bytesToRead);
        break;
        
    end
    
    if(countHeader==3 && buffer(k)==85)
        
        countHeader=4;
 
        if(bytesToRead-k > sizePayload)
            count =sizePayload;  
            frame(1:count) = buffer(k+1:k+sizePayload);  
            countBuffer =bytesToRead-k-sizePayload ; 
            buffer(1:countBuffer) = buffer(k+sizePayload+1:bytesToRead);
        else
            
            count =bytesToRead-k;
            if count > 0          
                frame(1:count) = buffer(k+1:bytesToRead);  
            end
            countBuffer = 0; 
            
        end
        
        break;
    end
    
    if(countHeader==2 && buffer(k)==102)
        countHeader=3;
    end
    
    if(countHeader==1 && buffer(k)==119)
        countHeader=2;
    end
       
    if(countHeader==0 && buffer(k)==136)
        countHeader=1;
    end

end

if count==sizePayload 
     frameOut = frame;
     flagOut = 1; 
     lastFrame = frame;
     frame=uint8(zeros(sizePayload,1));
     count=0;
     countHeader=0;
     
else % In case the buffer does not have an entire payload
    frameOut = lastFrame;
    flagOut = 0; 
end

== matlab function ARDroneTT/ARDrone Wi-Fi  Block/This block sets the heading angle to zero when the commands from the Simulink controller are enabled.  ==
  data: isFlying input; enableCmds input; yawOut output; yaw input
% Description: This function zeroes out the heading angle once the commands
% are enabled. 
function yawOut = fcn(isFlying,enableCmds,yaw)
%#codegen

yawOut = yaw; 
persistent yaw0 ; 
persistent mode ; 

if isempty (yaw0)
yaw0 = 0; 
end


if isempty (mode)
mode=0; 
end

if isFlying ==1 && enableCmds==1    
    yawOut = yaw - yaw0; 
    mode =1; 
elseif isFlying ==1 && mode ==0
    yaw0 = yaw; 
end


yawOut = mod(yawOut, 360) ;
if yawOut > 180
    yawOut = -360 + yawOut ; 
end

== matlab function ARDroneTT/MATLAB Function1 ==
  data: on_off input; states input; t input; pd output; dot_pd output; ddot_pd output; psi_d output; type output
function [pd, dot_pd, ddot_pd, psi_d, type] = desired_trajectory(on_off,states,t)
%#codegen

% ------------------------------------------------------------------------
% inputs:
% on_off - 1 if tracking is on, 0 if it is off
% states - structure with state variables
% t - current simulation time
% 
% outputs:
% pd - desired position
% dot_pd - desired velocity
% ddot_pd - desired acceleration
% psi_d - desired yaw angle
% ------------------------------------------------------------------------

persistent t0
persistent p0
persistent previous_status

on = 1;
off = 0;

if isempty(previous_status)
    previous_status = on;
    p0 = [states(7:8);-1];
end
type = -1;
if on_off == off
    if previous_status == on 
    % first time off or switching back off
        p0 = [states(7:8);-1]; % x0 and y0 match the current position
    end
    pd = p0;
    dot_pd = [0;0;0];
    ddot_pd = [0;0;0];
    psi_d = 0;
    type = -1;
else
    if isempty(t0) || (previous_status == off) 
    % first time on or switching back on
        t0 = t;
        p0 = [states(7:8);-1];
    end
    dt = t-t0;

%!!!!!!!!!!!!!!!!!!!!!!!!!!!!!!!!!!!!!!!!!!!!!!!!!!!!!!!!!!!!!!!!!!!!!!!!
% replace with the necessary code to define adequate desired trajectories
% use dt, p0, and any additional parameters (states is passed for the LOS planner)
    [pd, dot_pd, ddot_pd, psi_d, type] = desired_trajectory_self(dt, p0, states);
%!!!!!!!!!!!!!!!!!!!!!!!!!!!!!!!!!!!!!!!!!!!!!!!!!!!!!!!!!!!!!!!!!!!!!!!!

end

previous_status = on_off;

== matlab function ARDroneTT/Outer-loop Controller/Error Scopes/normalize angle between -pi and pi radians ==
  data: angleIn input; angleOut output
function angleOut = fcn(angleIn)
%#codegen

angleOut = mod(angleIn, 2*pi) ;
if angleOut > pi
    angleOut = -2*pi + angleOut ; 
end

== matlab function ARDroneTT/Outer-loop Controller/MATLAB Function ==
  data: w_r output; dot_psi_r output; theta_r output; states input; pd input; dot_pd input; ddot_pd input; psi_d input; xi input; phi_r output; dot_xi output
function [w_r, dot_psi_r, theta_r, phi_r, dot_xi] = tt_controller(states, pd, dot_pd, ddot_pd,psi_d,xi)

[w_r, dot_psi_r, theta_r, phi_r, dot_xi] = tt_controller_self(states, pd, dot_pd, ddot_pd,psi_d,xi);
end
